simulink model "GFMVSG1"  (R2024b)
settings: Solver=VariableStepAuto  StartTime=0.0  StopTime=20  RelTol=1e-3
undefined symbols (not defined in the file): sigbuilder_block
libraries: Model_DG_Grid_Forming_Converter x1, spsGroundLib x1, spsThreePhaseProgrammableVoltageSourceLib x1, spsThreePhaseSeriesRLCBranchLib x1, spsThreePhaseFaultLib x1, spspowerguiLib x1
settings Model: Creator=KIVANÇKOCAOĞULLAR  LastModifiedBy=KIVANÇKOCAOĞULLAR

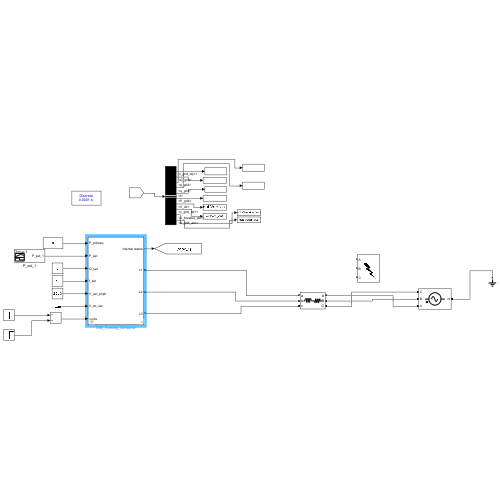
[thumbnail: Simulink's stored preview of the top-level diagram]
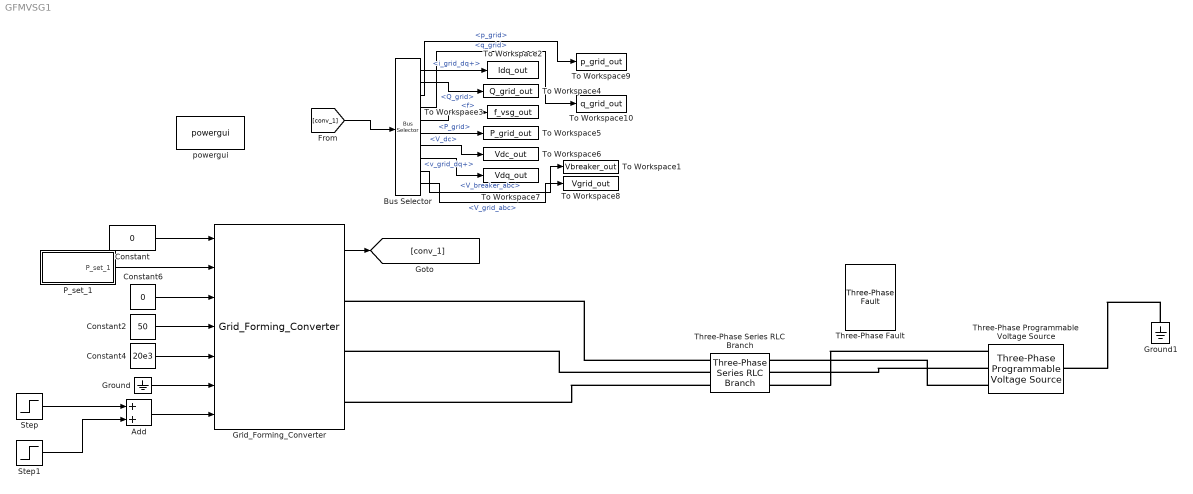
== system GFMVSG1 ==
  Add : Sum
  Bus Selector : BusSelector  OutputSignals=controller.measurements.dq+.i_grid_dq+,controller.measurements.Q_grid,controller.measurements.p_grid,controller.measurements.q_grid,controller.outer_control.f,controller.measurements.P_grid,physical.V_dc,controller.measurements.dq+.v_grid_dq+,physical.V_breaker_abc,physical.V_grid_abc
  Constant : Constant  Value=0
  Constant2 : Constant  Value=50
  Constant4 : Constant  Value=20e3
  Constant6 : Constant  Value=0
  Grid_Forming_Converter : Model_DG_Grid_Forming_Converter/Grid_Forming_Converter  S_n=2e6  V_n_phph=690  f_n=50  send_messages=on  T_s_ctrl=1e-4  T_s_PWM_meas=1e-4  T_s_SPS=1e-4  datatype='double'  swModeling=Average Model  f_sw=5e3  L_filter_conv_pu=[ 0.001 0.05097 ]  C_filter_pu=[ 0.06875 0.04569 ]  L_filter_grid_pu=[ 0.01 0.04 ]  C_dc_pu=0.75  withTransformer=Grid coupling using transformer  V_n_grid_phph=20e3  RL_Trafo_Conv=[ 0.005 0.02 ]  RL_Trafo_Grid=[ 0.005 0.02 ]  Rm=500  Lm=500  meas_lowpass=on  meas_f_cutoff_lowpass=2500  meas_f_cutoff_posseq=20  prot_variant=tDMSquared warnings only  v_dc_max=1.2  v_ac_max=1.4  t_ac_max=0.1  v_ac_maxmax=1.25  t_ac_maxmax=0.1  v_ac_min=0.8  t_ac_min=3  v_ac_minmin=0.45  t_ac_minmin=0.3  f_ac_max=51.5  t_f_ac_max=0.1  f_ac_maxmax=52.5  t_f_ac_maxmax=10  f_ac_min=47.5  t_f_ac_min=0.1  i_ac_max=1.3  outerCtrlStrategy=Virtual Synchronous Machine (VSM)  OuterCtrl_droop_kP=0.05  OuterCtrl_droop_kQ=0.1  OuterCtrl_droop_TQ=0.2  OuterCtrl_ZDroop_kf=0.05  OuterCtrl_ZDroop_kV=0.1  OuterCtrl_ZDroop_kR=0  OuterCtrl_ZDroop_kX=1  OuterCtrl_ZDroop_TV=0.2  OuterCtrl_VSM_H=3.4  OuterCtrl_VSM_Kd=5  OuterCtrl_VSM_K=20  OuterCtrl_VSM_kQ=0.1  OuterCtrl_VSM_TQ=0.2  OuterCtrl_Dual_Kp=0.01  OuterCtrl_Dual_Kd=1e-4  OuterCtrl_Dual_kQ=0.1  OuterCtrl_Dual_TQ=0.2  OuterCtrl_Lvirt=0  InnerCtrl_K_p_V_cap_controller=0.8  InnerCtrl_K_i_V_cap_controller=0.5  InnerCtrl_K_p_I_conv_controller=3.3  InnerCtrl_K_i_I_conv_controller=16.5  InnerCtrl_v_conv_max=1.3  InnerCtrl_i_conv_max=1.2  InnerCtrl_Cff_V_cap_ctrl=disabled  InnerCtrl_Cff_I_conv_ctrl=disabled  InnerCtrl_K_ff_I_grid=enabled  InnerCtrl_K_ff_V_cap=enabled  InnerCtrl_i_lim_type=dq coordinate system  InnerCtrl_active_damping=enabled  InnerCtrl_AD_R_virt_pu=0.2
      settings: SourceProductName=Grid-forming converter (3-phase)
  Ground : Ground
  Ground1 : spsGroundLib/Ground  LConnTagsString=a
  P_set_1 : Subsystem  Tag=STV Subsys  LoadFcn=sigbuilder_block('load');  StartFcn=sigbuilder_block('start');  StopFcn=sigbuilder_block('stop');  ClipboardFcn=sigbuilder_block('clipboard');  mask(Sigbuilder block){tuvar=[0:10]}
      mask help: Simulink:masks:SigbuilderBlock_MD
      mask init:
      | if ~strcmp(get_param(bdroot(gcbh),'SimulationStatus'),'stopped') tuvar = sigbuilder_block('maskInit'); end
      settings: CopyFcn=sigbuilder_block('copy');  DeleteFcn=sigbuilder_block('delete');  ModelCloseFcn=sigbuilder_block('modelClose');  PreSaveFcn=sigbuilder_block('preSave');  PauseFcn=sigbuilder_block('pause');  ContinueFcn=sigbuilder_block('continue');  NameChangeFcn=sigbuilder_block('namechange');  OpenFcn=sigbuilder_block('open',[-809.4 12.6 550.8 361.2 ]);  CloseFcn=sigbuilder_block('close');
      mask Display: plot(0, 0, 100, 100,[2, 2, 32, 32, 2], [68, 8, 8, 68, 68],[32, 2], [38, 38], [32, 19, 2],[53, 60, 44], [32, 17, 17, 2],[16, 16, 31, 31]);txt = getActiveGroup(gcbh);text(2, 100, txt,'verticalAlignment', 'top');
  Step : Step  Time=3  Before=-1  SampleTime=0
  Step1 : Step  Time=10  SampleTime=0
  Three-Phase Programmable Voltage Source : spsThreePhaseProgrammableVoltageSourceLib/Three-Phase Programmable Voltage Source  PositiveSequence=[20e3 0 50]  VariationEntity=None  VariationType=Table of time-amplitude pairs  VariationTypeAlt=Step  VariationStep=10  VariationRate=10  VariationMagnitude=0.3  VariationFrequency=2  VariationTiming=[15 100]  VariationPhaseA=off  Amplitudes=[1 0.8 1.2 1.0]  TimeValues=[0 0.1 0.15 0.2]  HarmonicGeneration=off  HarmonicA=[3 0.2 -25 0]  HarmonicB=[2 0.15 35 2]  Timing="[0.05  3]"  BusType=swing  Pref=0  Qref=0  Qmin=-inf  Qmax=inf
  Three-Phase Series RLC Branch : spsThreePhaseSeriesRLCBranchLib/Three-Phase Series RLC Branch  LConnTagsString=A|B|C  RConnTagsString=A|B|C  BranchType=RL  Resistance=3.98014876  Inductance=0.12669207  Capacitance=1e-6  Measurements=None
  Three-Phase Fault : spsThreePhaseFaultLib/Three-Phase Fault  InitialStates=0  FaultA=on  FaultB=on  FaultC=on  GroundFault=on  SwitchTimes=[100 101]  External=off  SwitchStatus=NaN  FaultResistance=0.001  GroundResistance=0.01  SnubberResistance=1e6  SnubberCapacitance=inf  Measurements=None
  To Workspace1 : ToWorkspace  VariableName=Vbreaker_out  SaveFormat=Timeseries  SampleTime=-1
  To Workspace10 : ToWorkspace  VariableName=q_grid_out  SaveFormat=Timeseries  SampleTime=-1
  To Workspace2 : ToWorkspace  VariableName=Idq_out  SaveFormat=Timeseries  SampleTime=-1
  To Workspace3 : ToWorkspace  VariableName=f_vsg_out  SaveFormat=Timeseries  SampleTime=-1
  To Workspace4 : ToWorkspace  VariableName=Q_grid_out  SaveFormat=Timeseries  SampleTime=-1
  To Workspace5 : ToWorkspace  VariableName=P_grid_out  SaveFormat=Timeseries  SampleTime=-1
  To Workspace6 : ToWorkspace  VariableName=Vdc_out  SaveFormat=Timeseries  SampleTime=-1
  To Workspace7 : ToWorkspace  VariableName=Vdq_out  SaveFormat=Timeseries  SampleTime=-1
  To Workspace8 : ToWorkspace  VariableName=Vgrid_out  SaveFormat=Timeseries  SampleTime=-1
  To Workspace9 : ToWorkspace  VariableName=p_grid_out  SaveFormat=Timeseries  SampleTime=-1
  powergui : spspowerguiLib/powergui  Priority=1  SimulationMode=Discrete  SampleTime=1e-4  frequency=60  Iterations=50  frequencyindice=50  Pbase=100e6  ErrMax=1e-4  UnitsV=kV  UnitsW=MW  buscounter=0  FunctionMessages=off  echomessages=off  EnableUseOfTLC=off  CurrentSourceSwitches=off  DisableSnubberDevices=off  DisableRonSwitches=off  DisableVfSwitches=off  DisplayEquations=off  AutomaticDiscreteSolvers=off  SolverType=Tustin/Backward Euler (TBE)  Interpol=off  ExternalGateDelay=off  methode=off  Ts=100  x0status=blocks  SPID=on  SwTol=0  HookPort=off  NonlinearTolerance=1e-4  nMaxIteration=100  ContinueOnMaxIteration=off  RestoreLinks=warning  ResistiveCurrentMeasurement=off  Frange=[0:2:500]  Ylog=off  Xlog=on  ShowGrid=off  save=off  variable=ZData  structure=0  ZoomFFT=off  StartTime=0.0  cycles=1  DisplayStyle=1  fundamental=60  FreqAxis=off  MaxFrequency=1000  frequencyindicesteady=1  RmsSteady=1  display=off
  wires:
  Step/1 -> Add/1
  Ground/1 -> Grid_Forming_Converter/6
  Add/1 -> Grid_Forming_Converter/7
  Grid_Forming_Converter/1 -> [conv_1]
  Constant6/1 -> Grid_Forming_Converter/3
  Constant/1 -> Grid_Forming_Converter/1
  Constant2/1 -> Grid_Forming_Converter/4
  Constant4/1 -> Grid_Forming_Converter/5
  Step1/1 -> Add/2
  [conv_1] -> Bus Selector/1
  Bus Selector/1 -> To Workspace2/1  "<i_grid_dq+>"
  Bus Selector/8 -> To Workspace7/1  "<v_grid_dq+>"
  Bus Selector/7 -> To Workspace6/1  "<V_dc>"
  Bus Selector/6 -> To Workspace5/1  "<P_grid>"
  Bus Selector/9 -> To Workspace1/1  "<V_breaker_abc>"
  Bus Selector/10 -> To Workspace8/1  "<V_grid_abc>"
  P_set_1/1(P_set_1) -> Grid_Forming_Converter/2
  Bus Selector/5 -> To Workspace3/1  "<f>"
  Bus Selector/2 -> To Workspace4/1  "<Q_grid>"
  Bus Selector/3 -> To Workspace9/1  "<p_grid>"
  Bus Selector/4 -> To Workspace10/1  "<q_grid>"
  connections:
  Ground1/LConn1 -- Three-Phase Programmable Voltage Source/LConn1
  Three-Phase Programmable Voltage Source/RConn2 -- Three-Phase Series RLC Branch/LConn2
  Three-Phase Programmable Voltage Source/RConn1 -- Three-Phase Series RLC Branch/LConn1
  Three-Phase Programmable Voltage Source/RConn3 -- Three-Phase Series RLC Branch/LConn3
  Three-Phase Series RLC Branch/RConn2 -- Grid_Forming_Converter/RConn2
  Three-Phase Series RLC Branch/RConn1 -- Grid_Forming_Converter/RConn1
  Three-Phase Series RLC Branch/RConn3 -- Grid_Forming_Converter/RConn3

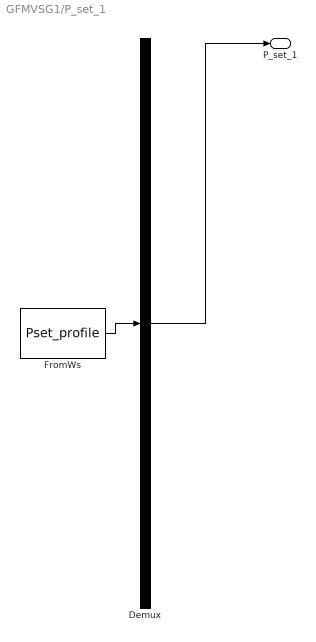
== system GFMVSG1/P_set_1 ==
  Demux : Demux  Tag=STV Demux  Outputs=1
      settings: DisplayOption=none
  FromWs : FromWorkspace  Tag=STV FromWs  VariableName=Pset_profile
      SigBuilderData=|
      | common.afterFinalStr = 'Extrapolate'
      | common.sampleTime = 0
      | dataSet.timeRange = [0 35]
      | dataSet.name = 'Group 1'
      | sbobj.Groups.Name = 'Group 1'
      | sbobj.Groups.Signals.Name = 'P_set_1'
      | sbobj.Groups.Signals.XData = [0 5 10 12 25 27 35]
      | sbobj.Groups.Signals.YData = [200000 200000 200000 700000 700000 800000 800000]
      | sbobj.Groups.TimeRange = [0 35]
  P_set_1 : Outport  Tag=STV Outport
  wires:
  Demux/1 -> P_set_1/1
  FromWs/1 -> Demux/1
